simulink model "QuadVisionControl_noise_delay"  (R2024a)
settings: Solver=ode4  StartTime=0.0  StopTime=30  FixedStep=0.005  RelTol=1e-3
InitFcn:
  | clear camera_delay_block_noise_160ms
undefined symbols (not defined in the file): idx
libraries: slpidlib x2, simulink x1
settings Model: Creator=Abbass  LastModifiedBy=Abbass
settings DataIOCC: ReturnWorkspaceOutputsName=out8

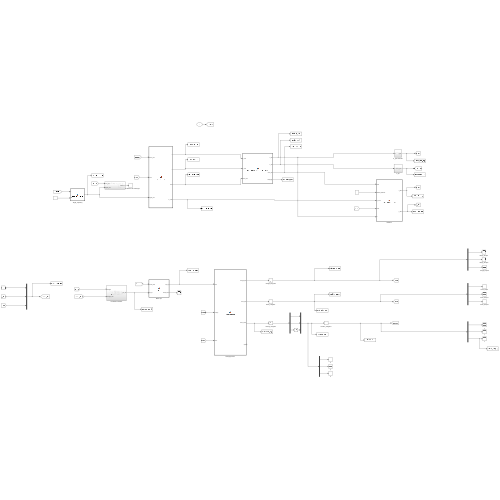
[thumbnail: Simulink's stored preview of the top-level diagram]
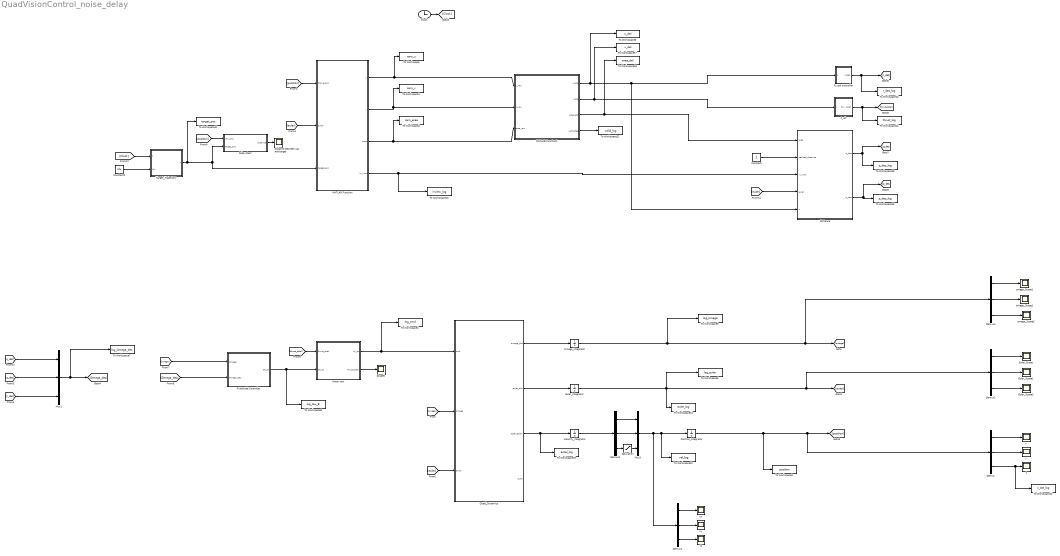
== system QuadVisionControl_noise_delay ==
  Clock : Clock
  Constant : Constant  Value=2
  Constant2 : Constant  Value=idx
  Demux{,1..4} (5 alike) : Demux  Outputs=3
  Distance : MATLAB Function  TreatAsAtomicUnit=on  SystemSampleTime=0.005
  Euler_Integrator : Integrator  InitialCondition=[0; 0; 2]
  Euler_Scope : Scope
  Euler_Scope1 : Scope
  Euler_Scope2 : Scope
  MATLAB Function : MATLAB Function  TreatAsAtomicUnit=on
  MATLAB Function1 : MATLAB Function  TreatAsAtomicUnit=on  SystemSampleTime=0.005
  Motor rpm : MATLAB Function  TreatAsAtomicUnit=on
  Mux1 : Mux  Inputs=3
  Mux3 : Mux  Inputs=3
  Omega_Integrator : Integrator
  PI attitude Controller : Subsystem
  P_alt : Subsystem
  P_yaw controller : Subsystem
  Position_Integrator : Integrator  InitialCondition=[15;5;7]
  Quad_Dynamics : MATLAB Function  TreatAsAtomicUnit=on
  Saturation : Saturate  UpperLimit=21  LowerLimit=-21
  Scope5 : Scope
  Subsystem : Subsystem
  Target_Trajectory : MATLAB Function  TreatAsAtomicUnit=on
  To Workspace : ToWorkspace  VariableName=cam_u  SampleTime=-1
  To Workspace1 : ToWorkspace  VariableName=cam_v  SampleTime=-1
  To Workspace10 : ToWorkspace  VariableName=euler_log  SampleTime=-1
  To Workspace11 : ToWorkspace  VariableName=target_pos  SampleTime=-1
  To Workspace12 : ToWorkspace  VariableName=z_sat_log  SaveFormat=Timeseries  SampleTime=-1
  To Workspace13 : ToWorkspace  VariableName=r_des_log  SaveFormat=Timeseries  SampleTime=-1
  To Workspace14 : ToWorkspace  VariableName=thrust_log  SaveFormat=Timeseries  SampleTime=-1
  To Workspace15 : ToWorkspace  VariableName=p_des_log  SaveFormat=Timeseries  SampleTime=-1
  To Workspace16 : ToWorkspace  VariableName=q_des_log  SaveFormat=Timeseries  SampleTime=-1
  To Workspace17 : ToWorkspace  VariableName=v_del  SampleTime=-1
  To Workspace18 : ToWorkspace  VariableName=area_del  SampleTime=-1
  To Workspace19 : ToWorkspace  VariableName=accel_log  SampleTime=-1
  To Workspace2 : ToWorkspace  VariableName=cam_area  SampleTime=-1
  To Workspace20 : ToWorkspace  VariableName=inview_log  SampleTime=-1
  To Workspace21 : ToWorkspace  VariableName=valid_log  SampleTime=-1
  To Workspace22 : ToWorkspace  VariableName=vel_log  SampleTime=-1
  To Workspace3 : ToWorkspace  VariableName=position  SampleTime=-1
  To Workspace4 : ToWorkspace  VariableName=log_cmd  SaveFormat=Timeseries  SampleTime=-1
  To Workspace5 : ToWorkspace  VariableName=log_euler  SaveFormat=Timeseries  SampleTime=-1
  To Workspace6 : ToWorkspace  VariableName=u_del  SampleTime=-1
  To Workspace7 : ToWorkspace  VariableName=log_Omega_des  SaveFormat=Timeseries  SampleTime=-1
  To Workspace8 : ToWorkspace  VariableName=log_tau_B  SaveFormat=Timeseries  SampleTime=-1
  To Workspace9 : ToWorkspace  VariableName=log_omega  SaveFormat=Timeseries  SampleTime=-1
  Velocity_Integrator : Integrator  InitialCondition=[0;0;0]
  "distance between uav and target " : Scope
  omega_Scope1 : Scope
  omega_Scope2 : Scope
  omega_Scope3 : Scope
  vx : Scope
  vy : Scope
  vz : Scope
  x : Scope
  y : Scope
  z : Scope
  wires:
  Quad_Dynamics/1(omega_dot) -> Omega_Integrator/1
  Quad_Dynamics/2(euler_dot) -> Euler_Integrator/1
  Quad_Dynamics/3(accel_earth) -> To Workspace19/1, Velocity_Integrator/1
  [euler] -> Quad_Dynamics/3(euler)
  [omega] -> Quad_Dynamics/2(omega)
  [Clock] -> Target_Trajectory/1(t)
  Constant2/1 -> Target_Trajectory/2(idx)
  Clock/1 -> [Clock]
  Target_Trajectory/1(T) -> To Workspace11/1, Subsystem/2(target_pos), MATLAB Function/3(target_pos)
  Position_Integrator/1 -> To Workspace3/1, Demux/1, [position]
  [position] -> MATLAB Function/1(drone_pos)
  [euler] -> MATLAB Function/2(euler)
  MATLAB Function/1(u) -> To Workspace/1, MATLAB Function1/1(u_raw)
  MATLAB Function/2(v) -> MATLAB Function1/2(v_raw), To Workspace1/1
  MATLAB Function/3(area) -> To Workspace2/1, MATLAB Function1/3(area_raw)
  Mux1/1 -> To Workspace7/1, [Omega_des]
  Distance/1(q_des) -> [q_des], To Workspace16/1
  [r_des] -> Mux1/3
  Motor rpm/1(Wi_sq) -> To Workspace4/1, Quad_Dynamics/1(cmd)
  [q_des] -> Mux1/2
  Euler_Integrator/1 -> To Workspace10/1, To Workspace5/1, Demux2/1, [euler]
  PI attitude Controller/1(tau_B) -> To Workspace8/1, Motor rpm/2(tau_B)
  [omega] -> PI attitude Controller/1(Omega)
  Demux/1 -> x/1
  Demux/2 -> y/1
  Demux/3 -> To Workspace12/1, z/1
  [thrust_total] -> Motor rpm/1("thrust_total ")
  [Omega_des] -> PI attitude Controller/2(Omega_des)
  Constant/1 -> Distance/2(desired_distance)
  [euler] -> Distance/4(euler)
  Demux2/1 -> Euler_Scope/1
  Demux2/2 -> Euler_Scope1/1
  Demux2/3 -> Euler_Scope2/1
  Velocity_Integrator/1 -> Demux3/1
  Demux4/3 -> omega_Scope3/1
  Demux4/2 -> omega_Scope2/1
  Demux4/1 -> omega_Scope1/1
  Omega_Integrator/1 -> To Workspace9/1, Demux4/1, [omega]
  Motor rpm/2(thrust_total) -> Scope5/1
  Distance/2(p_des) -> [p_des], To Workspace15/1
  Demux3/3 -> Saturation/1
  Subsystem/1(distance) -> "distance between uav and target "/1
  [position] -> Subsystem/1(uav_pos)
  [p_des] -> Mux1/1
  P_alt/1("thrust_total ") -> To Workspace14/1, [thrust_total]
  P_yaw controller/1(r_des) -> To Workspace13/1, [r_des]
  Demux3/1 -> Mux3/1
  Demux3/2 -> Mux3/2
  Saturation/1 -> Mux3/3
  Demux1/2 -> vy/1
  Demux1/1 -> vx/1
  Mux3/1 -> Demux1/1, To Workspace22/1, Position_Integrator/1
  Demux1/3 -> vz/1
  MATLAB Function1/1(u_del) -> To Workspace6/1, Distance/5(u), P_yaw controller/1(u)
  MATLAB Function1/2(v_del) -> To Workspace17/1, P_alt/1(v)
  MATLAB Function1/3(area_del) -> To Workspace18/1, Distance/1(area)
  MATLAB Function/4(in_view) -> To Workspace20/1, Distance/3(in_view)
  MATLAB Function1/4(valid_flag) -> To Workspace21/1

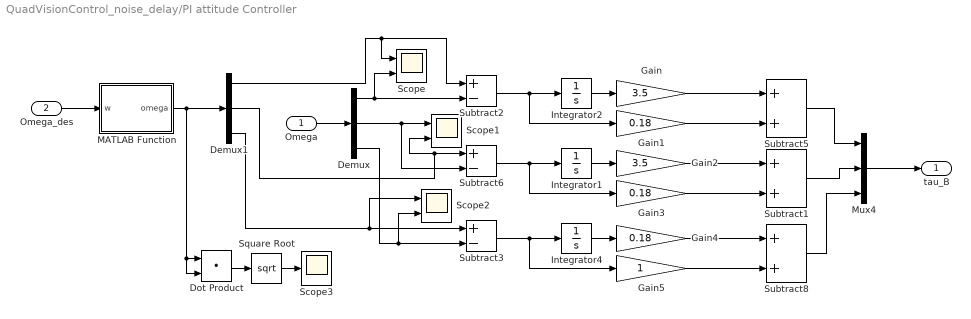
== system QuadVisionControl_noise_delay/PI attitude Controller ==
  Omega : Inport
  Omega_des : Inport  Port=2
  Demux : Demux  Outputs=3
  Demux1 : Demux  Outputs=3
  Dot Product : DotProduct  OutDataTypeStr=Inherit: Inherit via internal rule
  Gain : Gain  Gain=3.5
  Gain1 : Gain  Gain=0.18
  Gain2 : Gain  Gain=3.5
  Gain3 : Gain  Gain=0.18
  Gain4 : Gain  Gain=0.18
  Gain5 : Gain
  Integrator1 : Integrator
  Integrator2 : Integrator
  Integrator4 : Integrator
  MATLAB Function : MATLAB Function  TreatAsAtomicUnit=on
  Mux4 : Mux  Inputs=3
  Scope : Scope  NumInputPorts=2
  Scope1 : Scope  NumInputPorts=2
  Scope2 : Scope  NumInputPorts=2
  Scope3 : Scope
  Square Root : Sqrt
  Subtract1 : Sum
  Subtract2 : Sum  Inputs=+-
  Subtract3 : Sum  Inputs=+-
  Subtract5 : Sum
  Subtract6 : Sum  Inputs=+-
  Subtract8 : Sum
  tau_B : Outport
  wires:
  Gain5/1 -> Subtract8/2
  Gain1/1 -> Subtract5/2
  Subtract3/1 -> Gain5/1, Integrator4/1
  Integrator4/1 -> Gain4/1
  Subtract5/1 -> Mux4/1
  Gain4/1 -> Subtract8/1
  Integrator2/1 -> Gain/1
  Subtract2/1 -> Gain1/1, Integrator2/1
  Gain/1 -> Subtract5/1
  Subtract8/1 -> Mux4/3
  Mux4/1 -> tau_B/1
  Omega/1 -> Demux/1
  Demux/1 -> Scope/2, Subtract2/2
  Demux/2 -> Scope1/1, Subtract6/2
  Demux/3 -> Subtract3/2, Scope2/2
  Gain2/1 -> Subtract1/1
  Subtract6/1 -> Integrator1/1, Gain3/1
  Integrator1/1 -> Gain2/1
  Subtract1/1 -> Mux4/2
  Gain3/1 -> Subtract1/2
  MATLAB Function/1(omega) -> Demux1/1, Dot Product/2, Dot Product/1
  Dot Product/1 -> Square Root/1
  Square Root/1 -> Scope3/1
  Demux1/1 -> Scope/1, Subtract2/1
  Demux1/2 -> Scope1/2, Subtract6/1
  Demux1/3 -> Scope2/1, Subtract3/1
  Omega_des/1 -> MATLAB Function/1(w)

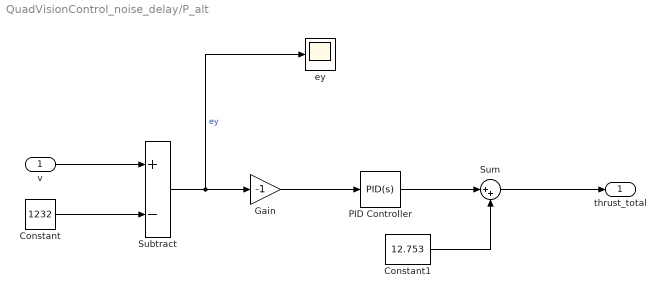
== system QuadVisionControl_noise_delay/P_alt ==
  v : Inport
  Constant : Constant  Value=1232
  Constant1 : Constant  Value=12.753
  Gain : Gain  Gain=-1
  PID Controller : slpidlib/PID Controller  Controller=PID  Form=Parallel  TimeDomain=Continuous-time  UseExternalTs=off  SampleTime=-1  IntegratorMethod=Forward Euler  FilterMethod=Forward Euler  ControllerParametersSource=internal  P=0.05  I=0.00  UseKiTs=off  D=0.1  UseExternalDerivativeSource=off  N=100  UseFilter=on  TunerSelectOption=Transfer Function Based (PID Tuner App)  InitialConditionSource=internal  InitialConditionForIntegrator=0  InitialConditionForFilter=0  DifferentiatorICPrevScaledInput=0  ExternalReset=none  TrackingMode=off  Kt=1  LimitOutput=off  SatLimitsSource=internal  UpperSaturationLimit=0.3  LowerSaturationLimit=-0.3  LinearizeAsGain=on  AntiWindupMode=none  Kb=1  LimitIntegrator=off  UpperIntegratorSaturationLimit=inf  LowerIntegratorSaturationLimit=-inf  POutMin=[]  POutMax=[]  IOutMin=[]  IOutMax=[]  DOutMin=[]  DOutMax=[]  NOutMin=[]  NOutMax=[]  SumOutMin=[]  SumOutMax=[]  SaturationOutMin=[]  SaturationOutMax=[]  PParamMin=[]  PParamMax=[]  IParamMin=[]  IParamMax=[]  DParamMin=[]  DParamMax=[]  NParamMin=[]  NParamMax=[]  KbParamMin=[]  KbParamMax=[]  KtParamMin=[]  KtParamMax=[]  KbOutMin=[]  KbOutMax=[]  KtOutMin=[]  KtOutMax=[]  IntegratorOutMin=[]  IntegratorOutMax=[]  FilterOutMin=[]  FilterOutMax=[]  SumI1OutMin=[]  SumI1OutMax=[]  SumI2OutMin=[]  SumI2OutMax=[]  SumI3OutMin=[]  SumI3OutMax=[]  SumI4OutMin=[]  SumI4OutMax=[]  SumDOutMin=[]  SumDOutMax=[]  DifferentiatorOutMin=[]  DifferentiatorOutMax=[]  FilterDiffOutCoefMin=[]  FilterDiffOutCoefMax=[]  ReciprocalOutMin=[]  ReciprocalOutMax=[]  SumDenOutMin=[]  SumDenOutMax=[]  SumNumOutMin=[]  SumNumOutMax=[]  DivideOutMin=[]  DivideOutMax=[]  UdiffTsProdOutMin=[]  UdiffTsProdOutMax=[]  NTsProdOutMin=[]  NTsProdOutMax=[]  UintegralTsProdOutMin=[]  UintegralTsProdOutMax=[]  UngainTsProdOutMin=[]  UngainTsProdOutMax=[]  ClampingZeroOutDataTypeStr=Inherit: Inherit via back propagation  ClampingZeroOutMin=[]  ClampingZeroOutMax=[]  FilterDenConstantOutDataTypeStr=Inherit: Inherit via back propagation  FilterDenConstantOutMin=[]  FilterDenConstantOutMax=[]  PCopyOutDataTypeStr=Inherit: Inherit via back propagation  PCopyOutMin=[]  PCopyOutMax=[]  NCopyOutDataTypeStr=Inherit: Inherit via back propagation  NCopyOutMin=[]  NCopyOutMax=[]  IntegratorContinuousStateAttributes=''  IntegratorStateMustResolveToSignalObject=off  IntegratorRTWStateStorageClass=Auto  FilterContinuousStateAttributes=''  FilterStateMustResolveToSignalObject=off  FilterRTWStateStorageClass=Auto  ParallelPVariant=InternalParameters  IdealPVariant=Disabled  IVariant=InternalParameters  DVariant=InternalParameters  IntegratorVariant=Continuous  SatVariant=Disabled  AWVariant=Passthrough  PCopyVariant=Disabled  TRVariant=Disabled  FdbkBlocksVariant=Forward  IdealPFdbkVariant=Disabled  SatFdbkVariant=Disabled  DerivativeFilterVariant=ContFilter  NVariant=InternalParameters  NCopyVariant=Disabled  FilterICVariant=InternalICsFilter  IntegratorICVariant=InternalICs  ExternalResetVariant=Disabled  TRSumVariant=Passthrough  SumFdbkVariant=Disabled  SumVariant=Sum_PID  TsampFilterVariant=InternalTs  TsampNgainVariant=Passthrough  TsampIntegralVariant=Disabled_SignalSpec  ExternalSaturationOutDataTypeStr=Inherit: Same as second input  DerivativeSourceVariant=ErrorSignal
  Subtract : Sum  Inputs=+-
  Sum : Sum  Inputs=|++
  ey : Scope
  "thrust_total " : Outport
  wires:
  Constant/1 -> Subtract/2
  v/1 -> Subtract/1
  Subtract/1 -> ey/1, Gain/1  "ey"
  Gain/1 -> PID Controller/1
  PID Controller/1 -> Sum/1
  Constant1/1 -> Sum/2
  Sum/1 -> "thrust_total "/1

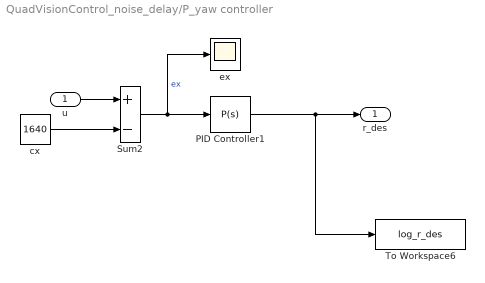
== system QuadVisionControl_noise_delay/P_yaw controller ==
  u : Inport
  PID Controller1 : slpidlib/PID Controller  Controller=P  Form=Parallel  TimeDomain=Continuous-time  UseExternalTs=off  SampleTime=-1  IntegratorMethod=Forward Euler  FilterMethod=Forward Euler  ControllerParametersSource=internal  P=-0.01  I=0  UseKiTs=off  D=0  UseExternalDerivativeSource=off  N=100  UseFilter=on  TunerSelectOption=Transfer Function Based (PID Tuner App)  InitialConditionSource=internal  InitialConditionForIntegrator=0  InitialConditionForFilter=0  DifferentiatorICPrevScaledInput=0  ExternalReset=none  TrackingMode=off  Kt=1  LimitOutput=off  SatLimitsSource=internal  UpperSaturationLimit=inf  LowerSaturationLimit=-inf  LinearizeAsGain=on  AntiWindupMode=none  Kb=1  LimitIntegrator=off  UpperIntegratorSaturationLimit=inf  LowerIntegratorSaturationLimit=-inf  POutMin=[]  POutMax=[]  IOutMin=[]  IOutMax=[]  DOutMin=[]  DOutMax=[]  NOutMin=[]  NOutMax=[]  SumOutMin=[]  SumOutMax=[]  SaturationOutMin=[]  SaturationOutMax=[]  PParamMin=[]  PParamMax=[]  IParamMin=[]  IParamMax=[]  DParamMin=[]  DParamMax=[]  NParamMin=[]  NParamMax=[]  KbParamMin=[]  KbParamMax=[]  KtParamMin=[]  KtParamMax=[]  KbOutMin=[]  KbOutMax=[]  KtOutMin=[]  KtOutMax=[]  IntegratorOutMin=[]  IntegratorOutMax=[]  FilterOutMin=[]  FilterOutMax=[]  SumI1OutMin=[]  SumI1OutMax=[]  SumI2OutMin=[]  SumI2OutMax=[]  SumI3OutMin=[]  SumI3OutMax=[]  SumI4OutMin=[]  SumI4OutMax=[]  SumDOutMin=[]  SumDOutMax=[]  DifferentiatorOutMin=[]  DifferentiatorOutMax=[]  FilterDiffOutCoefMin=[]  FilterDiffOutCoefMax=[]  ReciprocalOutMin=[]  ReciprocalOutMax=[]  SumDenOutMin=[]  SumDenOutMax=[]  SumNumOutMin=[]  SumNumOutMax=[]  DivideOutMin=[]  DivideOutMax=[]  UdiffTsProdOutMin=[]  UdiffTsProdOutMax=[]  NTsProdOutMin=[]  NTsProdOutMax=[]  UintegralTsProdOutMin=[]  UintegralTsProdOutMax=[]  UngainTsProdOutMin=[]  UngainTsProdOutMax=[]  ClampingZeroOutDataTypeStr=Inherit: Inherit via back propagation  ClampingZeroOutMin=[]  ClampingZeroOutMax=[]  FilterDenConstantOutDataTypeStr=Inherit: Inherit via back propagation  FilterDenConstantOutMin=[]  FilterDenConstantOutMax=[]  PCopyOutDataTypeStr=Inherit: Inherit via back propagation  PCopyOutMin=[]  PCopyOutMax=[]  NCopyOutDataTypeStr=Inherit: Inherit via back propagation  NCopyOutMin=[]  NCopyOutMax=[]  IntegratorContinuousStateAttributes=''  IntegratorStateMustResolveToSignalObject=off  IntegratorRTWStateStorageClass=Auto  FilterContinuousStateAttributes=''  FilterStateMustResolveToSignalObject=off  FilterRTWStateStorageClass=Auto  ParallelPVariant=InternalParameters  IdealPVariant=Disabled  IVariant=Disabled  DVariant=Disabled  IntegratorVariant=Disabled  SatVariant=Disabled  AWVariant=Disabled  PCopyVariant=Disabled  TRVariant=Disabled  FdbkBlocksVariant=Forward  IdealPFdbkVariant=Disabled  SatFdbkVariant=Disabled  DerivativeFilterVariant=Disabled  NVariant=Disabled  NCopyVariant=Disabled_SignalSpec  FilterICVariant=Disabled  IntegratorICVariant=Disabled  ExternalResetVariant=Disabled  TRSumVariant=Passthrough  SumFdbkVariant=Disabled  SumVariant=Passthrough_P  TsampFilterVariant=InternalTs  TsampNgainVariant=Passthrough  TsampIntegralVariant=Disabled_SignalSpec  ExternalSaturationOutDataTypeStr=Inherit: Same as second input  DerivativeSourceVariant=Disabled
  Sum2 : Sum  Inputs=+-
  To Workspace6 : ToWorkspace  VariableName=log_r_des  SaveFormat=Timeseries  SampleTime=-1
  cx : Constant  Value=1640
  ex : Scope
  r_des : Outport
  wires:
  u/1 -> Sum2/1
  cx/1 -> Sum2/2
  Sum2/1 -> ex/1, PID Controller1/1  "ex"
  PID Controller1/1 -> To Workspace6/1, r_des/1

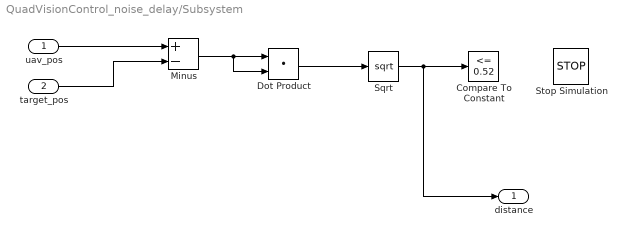
== system QuadVisionControl_noise_delay/Subsystem ==
  uav_pos : Inport
  target_pos : Inport  Port=2
  Compare To Constant : simulink/Logic and Bit Operations/Compare To Constant  relop=<=  const=0.52  OutDataTypeStr=boolean
  Dot Product : DotProduct  OutDataTypeStr=Inherit: Inherit via internal rule
  Minus : Sum  Inputs=+-
  Sqrt : Sqrt
  Stop Simulation : Stop
  distance : Outport
  wires:
  Dot Product/1 -> Sqrt/1
  Sqrt/1 -> distance/1, Compare To Constant/1
  Minus/1 -> Dot Product/1, Dot Product/2
  uav_pos/1 -> Minus/1
  target_pos/1 -> Minus/2

== matlab function QuadVisionControl_noise_delay/Target_Trajectory ==
  data: t input; T output; idx input
function T = target_trajectory_v2(t, idx)
%% TARGET_TRAJECTORY_V2 — Linear tracking scenarios (speed-matched to "normal UAV")
%
%  Speeds chosen so a normal quad (|Vx|,|Vy|~15 m/s, |Vz|~ few–20 m/s) can follow.
%
%  idx | Scenario              | Velocity
%  ----|-----------------------|------------------
%   1  | Stationary            | 0
%   2  | Climb Z               | Vz = 20 m/s
%   3  | Move -X               | Vx = -3 m/s
%   4  | Move +Y               | Vy =  3 m/s
%   5  | Y + Z                 | Vy = 5,  Vz = 20
%   6  | X + Y                 | Vx = 1,  Vy = 1
%   7  | X + Z                 | Vx = 1,  Vz = 20
%   8  | X + Y + Z             | Vx = 1,  Vy = 1, Vz = 20
%
%  In Simulink: replace target_trajectory with target_trajectory_v2
%  (same I/O: t, idx → T = [x; y; z])

    x = 0; y = 0; z = 0;

    switch idx
        case 1 % STATIONARY: fixed ahead
            x = 10; y = 0; z = 1;

        %% ── Vertical Tracking Tests (Moving Z) ──────────────
        case 2 % CLIMB: Target moves up at 20 m/s
            x = 10; y = 0;
            z = 1 + 20 * t;

        %% ── Horizontal Linear Tracking Tests ──────────────
        case 3 % MOVE -X: Target moves along -x at 3 m/s
            x = 10 - 3 * t;
            y = 0;
            z = 1;

        case 4 % MOVE +Y: Target moves along +y at 3 m/s
            x = 10;
            y = 3 * t;
            z = 1;

        %% ── Multi-Axis Linear Tracking Tests ──────────────
        case 5 % Y + Z: laterally and climbs
            x = 10;
            y = 5 * t;
            z = 1 + 20 * t;

        case 6 % X + Y: away and laterally
            x = 10 + 1 * t;
            y = 1 * t;
            z = 1;

        case 7 % X + Z: away and climbs
            x = 10 + 1 * t;
            y = 0;
            z = 1 + 20 * t;

        case 8 % X + Y + Z: all axes
            x = 10 + 1 * t;
            y = 1 * t;
            z = 1 + 20 * t;

        otherwise
            % Fallback: stationary
            x = 10; y = 0; z = 1;
    end

    T = [x; y; z];
end

== matlab function QuadVisionControl_noise_delay/Quad_Dynamics ==
  data: cmd input; omega_dot output; omega input; euler input; euler_dot output; accel_earth output; quat output
function [omega_dot, euler_dot, accel_earth, quat] = quad_dynamics(cmd, omega, euler)
%% QUAD_DYNAMICS — Complete 6-DOF quadrotor physics
%
%  INPUTS:
%    cmd   [4×1]  Motor commands (squared speeds ω² for each motor)
%    omega [3×1]  Current angular velocity [p; q; r] (rad/s)
%    euler [3×1]  Current Euler angles [φ; θ; ψ] (rad)
%
%  OUTPUTS:
%    omega_dot   [3×1]  Angular acceleration (rad/s²)
%    euler_dot   [3×1]  Euler angle rates (rad/s)
%    accel_earth [3×1]  Linear acceleration in Earth frame (m/s²)
%    quat        [4×1]  Quaternion [q0; q1; q2; q3] computed from Euler angles
%                       (needed by the Camera Model block)

%% ── Tell Simulink output sizes ─────────────────────────────
omega_dot   = zeros(3,1);
euler_dot   = zeros(3,1);
accel_earth = zeros(3,1);
quat        = zeros(4,1);

%% ── DRONE PARAMETERS (same as Quad_quat_control_v2) ─────────
m    = 1.3;            % mass (kg)
g    = 9.81;           % gravity (m/s²)
Ixx  = 0.0255;         % roll inertia (kg·m²)
Iyy  = 0.0255;         % pitch inertia (kg·m²)
Izz  = 0.0388;         % yaw inertia (kg·m²)
L    = 0.23;           % arm length center-to-motor (m)
kT   = 5e-6;           % thrust coefficient (N/(rad/s)²)
kQ   = 3e-7;           % torque coefficient (N·m/(rad/s)²)

%% ── STEP 1: Motor Model ────────────────────────────────────
T1 = kT * cmd(1);
T2 = kT * cmd(2);
T3 = kT * cmd(3);
T4 = kT * cmd(4);

%% ── STEP 2: Force & Torque Mixing ──────────────────────────
Fz = T1 + T2 + T3 + T4;
s45 = 0.7071;
tau_x = L * s45 * (T1 - T2 - T3 + T4);
tau_y = L * s45 * (T1 + T2 - T3 - T4);
tau_z = kQ * (-cmd(1) + cmd(2) - cmd(3) + cmd(4));

%% ── STEP 3: Extract current state ──────────────────────────
phi   = euler(1);
theta = euler(2);
psi   = euler(3);
p = omega(1);
q = omega(2);
r = omega(3);

%% ── STEP 4: Rotational Dynamics (Euler's Equation) ─────────
omega_dot(1) = (tau_x - (Izz - Iyy) * q * r) / Ixx;
omega_dot(2) = (tau_y - (Ixx - Izz) * p * r) / Iyy;
omega_dot(3) = (tau_z - (Iyy - Ixx) * p * q) / Izz;

%% ── STEP 5: Euler Angle Kinematics ─────────────────────────
euler_dot(1) = p + sin(phi)*tan(theta)*q + cos(phi)*tan(theta)*r;
euler_dot(2) = cos(phi)*q - sin(phi)*r;
euler_dot(3) = sin(phi)/cos(theta)*q + cos(phi)/cos(theta)*r;

%% ── STEP 6 & 7: Translational Dynamics + Rotation ──────────
ax_body = 0;
ay_body = 0;
az_body = Fz / m;

cphi = cos(phi);   sphi = sin(phi);
cth  = cos(theta); sth  = sin(theta);
cpsi = cos(psi);   spsi = sin(psi);

R11 = cpsi*cth;    R12 = cpsi*sth*sphi - spsi*cphi;   R13 = cpsi*sth*cphi + spsi*sphi;
R21 = spsi*cth;    R22 = spsi*sth*sphi + cpsi*cphi;   R23 = spsi*sth*cphi - cpsi*sphi;
R31 = -sth;        R32 = cth*sphi;                     R33 = cth*cphi;

accel_earth(1) = R11*ax_body + R12*ay_body + R13*az_body;
accel_earth(2) = R21*ax_body + R22*ay_body + R23*az_body;
accel_earth(3) = R31*ax_body + R32*ay_body + R33*az_body - g;

%% ── STEP 8: Euler → Quaternion (for Camera Model) ──────────
%  The old camera model uses quaternion (qNorm).
%  We compute it from Euler angles so we don't need a separate block.
%
%  Quaternion from ZYX Euler angles:
%    q = Rz(ψ) × Ry(θ) × Rx(φ)
%
%  Convention: q = [q0; q1; q2; q3] where q0 is the scalar part

cy = cos(psi/2);   sy = sin(psi/2);
cp = cos(theta/2); sp = sin(theta/2);
cr = cos(phi/2);   sr = sin(phi/2);

quat(1) = cr*cp*cy + sr*sp*sy;   % q0 (scalar)
quat(2) = sr*cp*cy - cr*sp*sy;   % q1 (x)
quat(3) = cr*sp*cy + sr*cp*sy;   % q2 (y)
quat(4) = cr*cp*sy - sr*sp*cy;   % q3 (z)

end

== matlab function QuadVisionControl_noise_delay/MATLAB Function ==
  data: drone_pos input; u output; euler input; target_pos input; v output; area output; in_view output
function [u, v, area, in_view] = camera_model(drone_pos, euler, target_pos)
%% CAMERA_MODEL — Pinhole camera projection
%
%  Simulates a forward-facing camera mounted on the drone.
%  Outputs the raw pixel coordinates (u, v) of the target.
%
%  INPUTS:
%    drone_pos  [3×1]  Drone position in Earth frame [x; y; z]
%    euler      [3×1]  Drone Euler angles [φ; θ; ψ] (rad)
%    target_pos [3×1]  Target position in Earth frame [x; y; z]
%
%  OUTPUTS:
%    u         scalar  Horizontal pixel coordinate of target in image
%    v         scalar  Vertical pixel coordinate of target in image
%    area      scalar  Target apparent area in pixels²
%    in_view   scalar  1 if target is visible, 0 if not
%
%  IMAGE CONVENTION:
%    (0, 0) = top-left corner
%    (cx, cy) = image center = (1640, 1232)
%    u increases to the RIGHT
%    v increases DOWNWARD
%
%  LATER: A delay block will sit AFTER this block.
%    Camera_Model → [u, v] → [Delay Block] → [u_del, v_del] → [Error Block]
%    Error block computes: px_error = u_del - cx, py_error = v_del - cy

%% ── Tell Simulink the output sizes ─────────────────────────
u       = 0;
v       = 0;
area    = 0;
in_view = 0;

%% ── CAMERA PARAMETERS ──────────────────────────────────────
img_width  = 3280;      % Image width (pixels)
img_height = 2464;      % Image height (pixels)
fov_h      = 160;       % Horizontal field of view (degrees)

% Focal length (pixels) calculated from FOV
fx = (img_width / 2) / tand(fov_h / 2);
fy = fx; % Assuming square pixels

% Image center (principal point)
cx = img_width  / 2;   % = 1640 pixels
cy = img_height / 2;   % = 1232 pixels

% Target physical radius (for area computation)
target_radius = 0.3;   % 30 cm radius

%% ── STEP 1: Relative position in Earth frame ───────────────
delta_earth = target_pos - drone_pos;

%% ── STEP 2: Rotation matrix (Earth → Body) ─────────────────
phi   = euler(1);
theta = euler(2);
psi   = euler(3);

cphi = cos(phi);   sphi = sin(phi);
cth  = cos(theta); sth  = sin(theta);
cpsi = cos(psi);   spsi = sin(psi);

% Earth-to-body rotation (transpose of body-to-earth)
Rb11 = cpsi*cth;     Rb12 = spsi*cth;     Rb13 = -sth;
Rb21 = cpsi*sth*sphi - spsi*cphi;  Rb22 = spsi*sth*sphi + cpsi*cphi;  Rb23 = cth*sphi;
Rb31 = cpsi*sth*cphi + spsi*sphi;  Rb32 = spsi*sth*cphi - cpsi*sphi;  Rb33 = cth*cphi;

%% ── STEP 3: Transform to body frame ────────────────────────
body_x = Rb11*delta_earth(1) + Rb12*delta_earth(2) + Rb13*delta_earth(3);
body_y = Rb21*delta_earth(1) + Rb22*delta_earth(2) + Rb23*delta_earth(3);
body_z = Rb31*delta_earth(1) + Rb32*delta_earth(2) + Rb33*delta_earth(3);

%% ── STEP 4: Check if target is in front of camera ──────────
if body_x < 0.1
    % Target is behind the drone or too close.
    % Tell the yaw controller which way to spin to find it!
    % body_y < 0 means target is to the RIGHT.
    if body_y < 0
        u = img_width; % Force maximum right error
    else
        u = 0;         % Force maximum left error
    end
    v       = cy;      % Keep pitch level while searching
    area    = 0;
    in_view = 0;
    return;
end

%% ── STEP 5: Pinhole projection (body → image pixels) ───────
%  Camera points along body x-axis (forward)
%  Image u (right) = body (-y)
%  Image v (down)  = body (-z)
u = fx * (-body_y / body_x) + cx;
v = fy * (-body_z / body_x) + cy;

%% ── STEP 6: Check if within image bounds ───────────────────
if u >= 0 && u <= img_width && v >= 0 && v <= img_height
    in_view = 1;
else
    % TARGET IS OUTSIDE THE FIELD OF VIEW!
    % A real camera cannot see it. Clamp u to the nearest edge
    % so the controller only knows "it went left" or "it went right"
    % but does NOT know the exact angle (no X-ray vision).
    u = max(0, min(img_width, u));
    v = max(0, min(img_height, v));
    area    = 0;
    in_view = 0;
end

%% ── STEP 7: Compute target apparent area ───────────────────
pixel_radius = fx * (target_radius / body_x);
area = pi * pixel_radius * pixel_radius;

%% ── STEP 8: Maximum Range Limit (Target too small) ───────────
% A real camera cannot detect a tiny spec at 1000 meters. 
% If the target is smaller than 16 pixels (about 2.2 px radius), it is LOST.
min_area_pixels = 16; 
if area < min_area_pixels && in_view == 1
    in_view = 0;
    % Leave u and v at the edge, the drone will enter "Search Mode"
end

end

== matlab function QuadVisionControl_noise_delay/Distance ==
  data: area input; desired_distance input; q_des output; in_view input; euler input; u input; p_des output
function [q_des, p_des] = distance_controller_v2(area, desired_distance, in_view, euler, u)
%% DISTANCE_CONTROLLER_V2 — Vision-Based Distance & Pitch Controller
%
%  PERFECT ZERO-DRIFT ARCHITECTURE:
%    1. Startup Yaw Gate:
%       Drone waits at t=0 until yaw controller rotates and centers the target
%       (u_error < 15 px ≈ 0.5°) before any forward pitch is allowed.
%       This guarantees zero lateral velocity (flies in a pure straight line).
%
%    2. Persistent Hover Lock:
%       Once aligned and active, the controller NEVER disconnects or shuts off.
%       It continuously holds 3.0m forever without time limits.
%
%    3. Overdamped Dead-Stop Braking:
%       Kp = 0.005, Kd = 0.06, max_angle = 0.035 rad (2.0° max tilt).
%
%  INPUTS:
%    area             [1×1]  Target apparent area (px²) from camera_model
%    desired_distance [1×1]  Desired distance from target (meters)
%    in_view          [1×1]  1 = target visible, 0 = lost
%    euler            [3×1]  Current Euler angles [phi; theta; psi] (rad)
%    u                [1×1]  Horizontal pixel of target from camera_model
%
%  OUTPUT:
%    q_des            [1×1]  Desired pitch rate (rad/s)

%% ── Camera parameters (MUST match camera_model.m!) ──────────
img_width     = 3280;
fov_h         = 160;       % degrees
fx            = (img_width / 2) / tand(fov_h / 2);
target_radius = 0.3;       % meters
cx            = img_width / 2;  % = 1640

%% ── Estimate current distance from area ─────────────────────
pixel_radius = sqrt(area / pi);
if pixel_radius > 0.1
    distance_est = fx * target_radius / pixel_radius;
else
    distance_est = 100;
end

%% ── Gains ───────────────────────────────────────────────────
DT = 0.005;
Kp_angle = 3.0;

%% ── Persistent states ───────────────────────────────────────
persistent prev_dist_err d_dist_filtered pitch_active prev_psi
if isempty(prev_dist_err)
    prev_dist_err   = 0;
    d_dist_filtered = 0;
    pitch_active    = 0;   % 0 = waiting for initial yaw alignment, 1 = active
    prev_psi        = euler(3);
end

%% ── Target lost → level immediately ─────────────────────────
if in_view < 0.5
    theta_current = euler(2);
    q_des = Kp_angle * (0 - theta_current);
    p_des = 5.0 * (0 - euler(1)); % Level the wings
    prev_dist_err   = 0;
    d_dist_filtered = 0;
    pitch_active    = 0;
    return;
end

%% ── Distance error ──────────────────────────────────────────
dist_error = distance_est - desired_distance;

%% ── INITIAL YAW ALIGNMENT GATE ──────────────────────────────
u_error = abs(u - cx);

% At startup: wait until yaw controller brings target to camera center (< 15 px)
if pitch_active == 0
    if u_error < 15
        pitch_active    = 1;
        prev_dist_err   = dist_error;
        d_dist_filtered = 0;
    end
end

%% ── CONTROL LAW ─────────────────────────────────────────────
theta_current = euler(2);

if pitch_active == 0
    %% ── STARTUP PHASE: Hold position & level while yaw aligns ─
    prev_dist_err   = dist_error;
    d_dist_filtered = 0;
    
    theta_des = 0;  % zero pitch until pointed directly at target
    q_des = Kp_angle * (theta_des - theta_current);
    
    % Level wings during startup
    phi_des = 0;
    p_des = 5.0 * (phi_des - euler(1));
    
else
    %% ── ACTIVE FLIGHT & INDEFINITE HOVER ────────────────────
    % Velocity damping filter
    d_dist_raw = (dist_error - prev_dist_err) / DT;
    prev_dist_err = dist_error;
    
    alpha = 0.10;  % Smoother filtering to prevent jitter
    d_dist_filtered = alpha * d_dist_raw + (1 - alpha) * d_dist_filtered;
    
    % Strictly enforce "Turn Before You Fly" to prevent sideways momentum and orbiting.
    % The camera is 160-deg FOV (fx=289). 30 pixels = ~6 degrees!
    % If the target is not almost perfectly centered, stop pitching.
    align_scale = max(0.0, min(1.0, 1.0 - (u_error - 10) / 20));
    
    % ── DUAL-MODE CONTROLLER ──
    e_abs = abs(dist_error);
    
    % Mode 1: Fast Cinematic Approach (Square-root profile for early braking)
    V_des = sign(dist_error) * min(3.0, sqrt(2 * 0.4 * e_abs));
    V_actual = -d_dist_filtered;
    theta_approach = 0.15 * (V_des - V_actual);
    
    % Mode 2: Snappy, Critically Damped Settling
    % Kp=0.04, Kd=0.12 gives a perfect zeta=1.0 damping ratio (no creeping, no bouncing)
    theta_settle = 0.04 * dist_error + 0.12 * d_dist_filtered;
    
    % Smooth blending based on distance
    % > 2.0m = 100% Approach, < 0.5m = 100% Settle
    blend_factor = max(0, min(1, (e_abs - 0.5) / 1.5));
    
    theta_des = align_scale * (blend_factor * theta_approach + (1 - blend_factor) * theta_settle);
    
    % Safe tilt limit: ±6.8 degrees (0.12 rad)
    max_angle = 0.12;
    theta_des = max(-max_angle, min(max_angle, theta_des));
    
    % Inner loop P control
    q_des = Kp_angle * (theta_des - theta_current);
    
    %% ── ACTIVE LATERAL BRAKING (ROLL CONTROL) ───────────────────
    % The drone was orbiting because the Yaw controller kept the target
    % perfectly centered, so u_error was 0.
    % However, if the drone is orbiting, it is CONSTANTLY yawing!
    % We calculate the yaw rate, and bank (roll) into the turn to stop it.
    
    % Safely calculate yaw rate (handling -pi to pi wrap-around)
    d_psi = euler(3) - prev_psi;
    if d_psi > pi,  d_psi = d_psi - 2*pi; end
    if d_psi < -pi, d_psi = d_psi + 2*pi; end
    yaw_rate = d_psi / DT;
    prev_psi = euler(3);
    
    % Base visual servoing
    phi_vis = 0.0012 * u_error; 
    if u < cx, phi_vis = -phi_vis; end
    
    % Active Orbit Damping (Bank into the turn)
    % If yawing left (yaw_rate > 0), bank left (phi < 0).
    phi_damp = -0.15 * yaw_rate;
    
    phi_des = phi_vis + phi_damp;
    
    % Safe bank limit: ±25 degrees (0.43 rad)
    max_bank = 0.43;
    phi_des = max(-max_bank, min(max_bank, phi_des));
    
    % Inner loop Roll P control
    p_des = 5.0 * (phi_des - euler(1));
end

%% ── Limit angular rates ────────────────────────────────────────
max_pitch_rate = 0.2;
max_roll_rate  = 0.5;

q_des = max(-max_pitch_rate, min(max_pitch_rate, q_des));
p_des = max(-max_roll_rate, min(max_roll_rate, p_des));

end

== matlab function QuadVisionControl_noise_delay/MATLAB Function1 ==
  data: u_raw input; u_del output; v_raw input; area_raw input; v_del output; area_del output; valid_flag output
function [u_del, v_del, area_del, valid_flag] = camera_delay_block_noise_160ms(u_raw, v_raw, area_raw)
%#codegen
%CAMERA_DELAY_BLOCK_NOISE_160MS  Imaging delay 160 ms + detector noise
%
%  Identical to camera_delay_block_with_area_160ms EXCEPT that measurement
%  noise is added at the instant a new frame is latched. This completes the
%  measurement model of Yang et al. Eq. (11), which the noise-free block
%  quotes but does not implement:
%
%       i_p_img,k = i_p_{k-D} + n_img
%                                ^^^^^  <-- this term
%
%  WHY THE NOISE GOES HERE, NOT IN camera_model.m
%    - camera_model.m stays byte-identical, so out1..out5 remain exactly
%      reproducible and the old models never have to be re-run.
%    - Noise is drawn ONCE PER CAMERA FRAME (~30 Hz), not once per 5 ms
%      control step. A detector produces one estimate per image; holding it
%      between frames is the physically correct behaviour.
%    - The undelayed camera output stays clean, so it is still usable as
%      ground truth when scoring the observers.
%
%  NOISE MODEL
%    u, v  : additive Gaussian, sigma = SIGMA_UV pixels (centroid jitter)
%    area  : noise applied to the apparent RADIUS, not the area, then
%            squared back. Radius ~ 1/range with roughly constant pixel
%            noise, whereas area ~ 1/range^2 with noise scaling as
%            range^4 - adding noise to area directly would be unphysical
%            and would wreck the DKF covariance at long range.
%    Consequence, by design: range noise GROWS with distance. At 10 m the
%    blob radius is ~8.7 px so 0.25 px is ~2.9% -> ~0.29 m of range error;
%    at 2 m the radius is ~43 px so the same 0.25 px is ~0.6% -> ~1.2 cm.
%    This is the real reason an adaptive gain can beat a fixed one.
%
%  DETERMINISM  (this is what makes out6 vs out7 a fair comparison)
%    A self-contained linear congruential generator with an explicit seed is
%    used instead of randn, so the noise sequence does NOT depend on
%    MATLAB's global random stream, on block execution order, or on which
%    model is running. Paste this same body into BOTH new models and they
%    draw the identical sequence.
%
%    NOTE: in closed loop the two aircraft still diverge, so the same noise
%    numbers land on different true values. That is unavoidable and is not a
%    fairness problem - what matters is that neither run got a luckier draw.
%
%  REQUIRED SETUP
%    1. MATLAB Function block sample time = 0.005 (same as the old block).
%    2. Add to the model InitFcn, alongside the existing clear lines:
%           clear camera_delay_block_noise_160ms
%       Without this the persistent RNG state survives between runs and run
%       N+1 will not reproduce run N.
%    3. Use the SAME seed in both new models. Do not "vary it for realism".

    %% == Timing constants (unchanged from the noise-free block) ==========
    DT_IMU   = 0.005;                      % 200 Hz control/IMU step
    DT_CAM   = 1/30;                       % ~30 Hz camera frame rate
    DELAY_S  = 0.160;                      % 160 ms imaging+processing delay

    D_STEPS  = round(DELAY_S / DT_IMU);    % 32 steps = 160 ms
    CAM_STEP = round(DT_CAM  / DT_IMU);    % 7 steps ~= 30 Hz camera period
    BUF_LEN  = D_STEPS + 2;

    %% == Noise constants =================================================
    SIGMA_UV  = 1.5;        % px, centroid jitter (both axes)
    SIGMA_S   = 0.25;       % px, apparent-radius jitter
    NOISE_SEED = 12345;     % identical in both models. Do not change.

    IMG_W = 3280;           % clamp bounds, must match camera_model.m
    IMG_H = 2464;

    %% == Persistent state ================================================
    persistent step_count u_buf v_buf area_buf buf_idx p_held initialized rng_state

    if isempty(initialized)
        step_count  = 0;
        u_buf       = zeros(BUF_LEN, 1);
        v_buf       = zeros(BUF_LEN, 1);
        area_buf    = zeros(BUF_LEN, 1);
        buf_idx     = 0;
        p_held      = [0; 0; 0];
        rng_state   = NOISE_SEED;
        initialized = true;
    end

    step_count = step_count + 1;

    %% == Store the current (true, undelayed, CLEAN) reading ==============
    buf_idx = buf_idx + 1;
    if buf_idx > BUF_LEN
        buf_idx = 1;
    end
    u_buf(buf_idx)    = u_raw;
    v_buf(buf_idx)    = v_raw;
    area_buf(buf_idx) = area_raw;

    %% == Warm start ======================================================
    if step_count == 1
        p_held = [u_raw; v_raw; area_raw];
    end

    %% == Camera trigger (~30 Hz): fetch sample from D_STEPS ago, ADD NOISE
    valid_flag = double(0);
    if mod(step_count - 1, CAM_STEP) == 0
        if step_count > D_STEPS
            src_idx = buf_idx - D_STEPS;
            if src_idx < 1
                src_idx = src_idx + BUF_LEN;   % circular wrap
            end

            u_t = u_buf(src_idx);
            v_t = v_buf(src_idx);
            a_t = area_buf(src_idx);

            % --- draw three independent N(0,1) samples ------------------
            [g1, rng_state] = local_randn(rng_state);
            [g2, rng_state] = local_randn(rng_state);
            [g3, rng_state] = local_randn(rng_state);

            % --- centroid noise -----------------------------------------
            u_n = u_t + SIGMA_UV * g1;
            v_n = v_t + SIGMA_UV * g2;
            u_n = max(0, min(IMG_W, u_n));
            v_n = max(0, min(IMG_H, v_n));

            % --- radius noise, only when the target is actually seen -----
            % area_raw = 0 means not in view. Never manufacture a detection
            % out of noise: leave it at 0 so the observer's min_area gate
            % correctly rejects the frame.
            if a_t > 1e-9
                s_t = sqrt(a_t / pi);
                s_n = s_t + SIGMA_S * g3;
                if s_n < 0.5
                    s_n = 0.5;           % a blob cannot be sub-pixel
                end
                a_n = pi * s_n * s_n;
            else
                a_n = 0;
            end

            p_held     = [u_n; v_n; a_n];
            valid_flag = double(1);
        end
    end

    %% == Output: sample-and-hold noisy delayed measurement ===============
    u_del    = p_held(1);
    v_del    = p_held(2);
    area_del = p_held(3);

end


%% ---------------------------------------------------------------------
function [g, s] = local_randn(s)
%  One N(0,1) sample via Box-Muller from a deterministic LCG.
%  Numerical note: the LCG multiply reaches ~6.7e15, safely inside the
%  2^53 exact-integer range of double, so this is bit-reproducible.
[u1, s] = local_rand(s);
[u2, s] = local_rand(s);
if u1 < 1e-12
    u1 = 1e-12;                 % guard log(0)
end
g = sqrt(-2*log(u1)) * cos(2*pi*u2);
end


function [u, s] = local_rand(s)
%  Numerical Recipes LCG, period 2^32.
s = mod(1664525*s + 1013904223, 4294967296);
u = (s + 0.5) / 4294967296;     % strictly inside (0,1)
end

== matlab function QuadVisionControl_noise_delay/Motor rpm ==
  data: thrust_total input; Wi_sq output; tau_B input; thrust_total output
function [Wi_sq, thrust_total] = fcn(thrust_total, tau_B)
    % Quadrotor Parameters (same as Quad_quat_control_v2)
    Kf = 5e-6;           % Thrust coefficient (N/(rad/s)^2)
    Kt = 3e-7;           % Reaction Torque coefficient (N·m/(rad/s)^2)
    L  = 0.23;           % Length of the arm (m)
    m  = 1.3;            % Mass of the quadrotor (kg)
    g  = 9.81;           % Gravity (m/s^2)

    % Extract torques from tau_B vector
    Troll  = tau_B(1);
    Tpitch = tau_B(2);
    Tyaw   = tau_B(3);

    % Saturate total thrust (max = 60N, same as original)
    thrust_total = max(0, min(thrust_total, 60));

    %*****************************************************************
    % % Motors Speeds
    % Sign convention matches quad_dynamics.m:
    %   tau_x = L*s45*kT*( w1^2 - w2^2 - w3^2 + w4^2)
    %   tau_y = L*s45*kT*( w1^2 + w2^2 - w3^2 - w4^2)
    %   tau_z = Kt     *(-w1^2 + w2^2 - w3^2 + w4^2)

    s2 = sqrt(2);

    W1_sq = max(0, (1/4)*(thrust_total/Kf + s2*Troll/(L*Kf) + s2*Tpitch/(L*Kf) - Tyaw/Kt));
    W2_sq = max(0, (1/4)*(thrust_total/Kf - s2*Troll/(L*Kf) + s2*Tpitch/(L*Kf) + Tyaw/Kt));
    W3_sq = max(0, (1/4)*(thrust_total/Kf - s2*Troll/(L*Kf) - s2*Tpitch/(L*Kf) - Tyaw/Kt));
    W4_sq = max(0, (1/4)*(thrust_total/Kf + s2*Troll/(L*Kf) - s2*Tpitch/(L*Kf) + Tyaw/Kt));

    Wi_sq = [W1_sq W2_sq W3_sq W4_sq];
end

== matlab function QuadVisionControl_noise_delay/PI attitude Controller/MATLAB Function ==
  data: w input; omega output
function omega = saturation(w)
if norm(w)>6.283
   omega= 6.283*w/norm(w);
else omega=w;
end
